simulink model "MMC_Rectifier_NLM_2018"  (R2023b)
settings: Solver=ode23t  StartTime=0.0  StopTime=3  RelTol=1e-3
libraries: spsIGBTDiodeLib x216, spsSeriesRLCBranchLib x117, spsVoltageMeasurementLib x110, spsCurrentMeasurementLib x7, slpidlib x6, spsThreePhaseVIMeasurementLib x2, spsGroundLib x1, spsPower3phInstantaneousLib x1, spsThreePhaseProgrammableVoltageSourceLib x1, spsThreePhaseSeriesRLCBranchLib x1, spspowerguiLib x1
(part 3 of 5)

== system MMC_Rectifier_NLM_2018/MMC  Rectifier/MMC1/MMC7 ==
  PWM : Inport
  IGBT/Diode : spsIGBTDiodeLib/IGBT//Diode  Ron=1e-3  Rs=1e5  Cs=inf  Measurements=off
  IGBT/Diode1 : spsIGBTDiodeLib/IGBT//Diode  Ron=1e-3  Rs=1e5  Cs=inf  Measurements=off
  Logical Operator : Logic  Inputs=1  AllPortsSameDT=off  OutDataTypeStr=boolean
  Logical Operator1 : Logic  Operator=NOT  Inputs=1  AllPortsSameDT=off  OutDataTypeStr=boolean
  Series RLC Branch : spsSeriesRLCBranchLib/Series RLC Branch  LConnTagsString=__new0  RConnTagsString=__new0  BranchType=C  Resistance=1  Inductance=1e-3  SetiL0=off  InitialCurrent=0  Capacitance=C0  Setx0=on  InitialVoltage=V0  Measurements=None
  Voltage Measurement : spsVoltageMeasurementLib/Voltage Measurement  PhasorSimulation=off  OutputType=Complex  PSBequivalent=0
  V+ : PMIOPort  Side=Left
  V- : PMIOPort  Port=2  Side=Left
  VC : Outport
  wires:
  Logical Operator1/1 -> IGBT/Diode1/1
  Voltage Measurement/1 -> VC/1
  Logical Operator/1 -> IGBT/Diode/1
  PWM/1 -> Logical Operator/1, Logical Operator1/1
  connections:
  Voltage Measurement/LConn1 -- Series RLC Branch/LConn1 -- IGBT/Diode/LConn1
  V+/RConn1 -- IGBT/Diode1/LConn1 -- IGBT/Diode/RConn1
  V-/RConn1 -- IGBT/Diode1/RConn1 -- Series RLC Branch/RConn1 -- Voltage Measurement/LConn2

== system MMC_Rectifier_NLM_2018/MMC  Rectifier/MMC1/MMC8 ==
  PWM : Inport
  IGBT/Diode : spsIGBTDiodeLib/IGBT//Diode  Ron=1e-3  Rs=1e5  Cs=inf  Measurements=off
  IGBT/Diode1 : spsIGBTDiodeLib/IGBT//Diode  Ron=1e-3  Rs=1e5  Cs=inf  Measurements=off
  Logical Operator : Logic  Inputs=1  AllPortsSameDT=off  OutDataTypeStr=boolean
  Logical Operator1 : Logic  Operator=NOT  Inputs=1  AllPortsSameDT=off  OutDataTypeStr=boolean
  Series RLC Branch : spsSeriesRLCBranchLib/Series RLC Branch  LConnTagsString=__new0  RConnTagsString=__new0  BranchType=C  Resistance=1  Inductance=1e-3  SetiL0=off  InitialCurrent=0  Capacitance=C0  Setx0=on  InitialVoltage=V0  Measurements=None
  Voltage Measurement : spsVoltageMeasurementLib/Voltage Measurement  PhasorSimulation=off  OutputType=Complex  PSBequivalent=0
  V+ : PMIOPort  Side=Left
  V- : PMIOPort  Port=2  Side=Left
  VC : Outport
  wires:
  Logical Operator1/1 -> IGBT/Diode1/1
  Voltage Measurement/1 -> VC/1
  Logical Operator/1 -> IGBT/Diode/1
  PWM/1 -> Logical Operator/1, Logical Operator1/1
  connections:
  Voltage Measurement/LConn1 -- Series RLC Branch/LConn1 -- IGBT/Diode/LConn1
  V+/RConn1 -- IGBT/Diode1/LConn1 -- IGBT/Diode/RConn1
  V-/RConn1 -- IGBT/Diode1/RConn1 -- Series RLC Branch/RConn1 -- Voltage Measurement/LConn2

== system MMC_Rectifier_NLM_2018/MMC  Rectifier/MMC1/MMC9 ==
  PWM : Inport
  IGBT/Diode : spsIGBTDiodeLib/IGBT//Diode  Ron=1e-3  Rs=1e5  Cs=inf  Measurements=off
  IGBT/Diode1 : spsIGBTDiodeLib/IGBT//Diode  Ron=1e-3  Rs=1e5  Cs=inf  Measurements=off
  Logical Operator : Logic  Inputs=1  AllPortsSameDT=off  OutDataTypeStr=boolean
  Logical Operator1 : Logic  Operator=NOT  Inputs=1  AllPortsSameDT=off  OutDataTypeStr=boolean
  Series RLC Branch : spsSeriesRLCBranchLib/Series RLC Branch  LConnTagsString=__new0  RConnTagsString=__new0  BranchType=C  Resistance=1  Inductance=1e-3  SetiL0=off  InitialCurrent=0  Capacitance=C0  Setx0=on  InitialVoltage=V0  Measurements=None
  Voltage Measurement : spsVoltageMeasurementLib/Voltage Measurement  PhasorSimulation=off  OutputType=Complex  PSBequivalent=0
  V+ : PMIOPort  Side=Left
  V- : PMIOPort  Port=2  Side=Left
  VC : Outport
  wires:
  PWM/1 -> Logical Operator1/1, Logical Operator/1
  Logical Operator/1 -> IGBT/Diode/1
  Voltage Measurement/1 -> VC/1
  Logical Operator1/1 -> IGBT/Diode1/1
  connections:
  Voltage Measurement/LConn2 -- Series RLC Branch/RConn1 -- IGBT/Diode1/RConn1 -- V-/RConn1
  IGBT/Diode/RConn1 -- IGBT/Diode1/LConn1 -- V+/RConn1
  IGBT/Diode/LConn1 -- Series RLC Branch/LConn1 -- Voltage Measurement/LConn1

== system MMC_Rectifier_NLM_2018/MMC  Rectifier/MMC2/MMC ==
  PWM : Inport
  IGBT/Diode : spsIGBTDiodeLib/IGBT//Diode  Ron=1e-3  Rs=1e5  Cs=inf  Measurements=off
  IGBT/Diode1 : spsIGBTDiodeLib/IGBT//Diode  Ron=1e-3  Rs=1e5  Cs=inf  Measurements=off
  Logical Operator : Logic  Inputs=1  AllPortsSameDT=off  OutDataTypeStr=boolean
  Logical Operator1 : Logic  Operator=NOT  Inputs=1  AllPortsSameDT=off  OutDataTypeStr=boolean
  Series RLC Branch : spsSeriesRLCBranchLib/Series RLC Branch  LConnTagsString=__new0  RConnTagsString=__new0  BranchType=C  Resistance=1  Inductance=1e-3  SetiL0=off  InitialCurrent=0  Capacitance=C0  Setx0=on  InitialVoltage=V0  Measurements=None
  Voltage Measurement : spsVoltageMeasurementLib/Voltage Measurement  PhasorSimulation=off  OutputType=Complex  PSBequivalent=0
  V+ : PMIOPort  Side=Left
  V- : PMIOPort  Port=2  Side=Left
  VC : Outport
  wires:
  PWM/1 -> Logical Operator1/1, Logical Operator/1
  Logical Operator/1 -> IGBT/Diode/1
  Voltage Measurement/1 -> VC/1
  Logical Operator1/1 -> IGBT/Diode1/1
  connections:
  Series RLC Branch/RConn1 -- Voltage Measurement/LConn2 -- V-/RConn1 -- IGBT/Diode1/RConn1
  IGBT/Diode1/LConn1 -- V+/RConn1 -- IGBT/Diode/RConn1
  Series RLC Branch/LConn1 -- Voltage Measurement/LConn1 -- IGBT/Diode/LConn1

== system MMC_Rectifier_NLM_2018/MMC  Rectifier/MMC2/MMC1 ==
  PWM : Inport
  IGBT/Diode : spsIGBTDiodeLib/IGBT//Diode  Ron=1e-3  Rs=1e5  Cs=inf  Measurements=off
  IGBT/Diode1 : spsIGBTDiodeLib/IGBT//Diode  Ron=1e-3  Rs=1e5  Cs=inf  Measurements=off
  Logical Operator : Logic  Inputs=1  AllPortsSameDT=off  OutDataTypeStr=boolean
  Logical Operator1 : Logic  Operator=NOT  Inputs=1  AllPortsSameDT=off  OutDataTypeStr=boolean
  Series RLC Branch : spsSeriesRLCBranchLib/Series RLC Branch  LConnTagsString=__new0  RConnTagsString=__new0  BranchType=C  Resistance=1  Inductance=1e-3  SetiL0=off  InitialCurrent=0  Capacitance=C0  Setx0=on  InitialVoltage=V0  Measurements=None
  Voltage Measurement : spsVoltageMeasurementLib/Voltage Measurement  PhasorSimulation=off  OutputType=Complex  PSBequivalent=0
  V+ : PMIOPort  Side=Left
  V- : PMIOPort  Port=2  Side=Left
  VC : Outport
  wires:
  Logical Operator1/1 -> IGBT/Diode1/1
  Voltage Measurement/1 -> VC/1
  Logical Operator/1 -> IGBT/Diode/1
  PWM/1 -> Logical Operator/1, Logical Operator1/1
  connections:
  Voltage Measurement/LConn1 -- Series RLC Branch/LConn1 -- IGBT/Diode/LConn1
  V+/RConn1 -- IGBT/Diode1/LConn1 -- IGBT/Diode/RConn1
  V-/RConn1 -- IGBT/Diode1/RConn1 -- Series RLC Branch/RConn1 -- Voltage Measurement/LConn2

== system MMC_Rectifier_NLM_2018/MMC  Rectifier/MMC2/MMC10 ==
  PWM : Inport
  IGBT/Diode : spsIGBTDiodeLib/IGBT//Diode  Ron=1e-3  Rs=1e5  Cs=inf  Measurements=off
  IGBT/Diode1 : spsIGBTDiodeLib/IGBT//Diode  Ron=1e-3  Rs=1e5  Cs=inf  Measurements=off
  Logical Operator : Logic  Inputs=1  AllPortsSameDT=off  OutDataTypeStr=boolean
  Logical Operator1 : Logic  Operator=NOT  Inputs=1  AllPortsSameDT=off  OutDataTypeStr=boolean
  Series RLC Branch : spsSeriesRLCBranchLib/Series RLC Branch  LConnTagsString=__new0  RConnTagsString=__new0  BranchType=C  Resistance=1  Inductance=1e-3  SetiL0=off  InitialCurrent=0  Capacitance=C0  Setx0=on  InitialVoltage=V0  Measurements=None
  Voltage Measurement : spsVoltageMeasurementLib/Voltage Measurement  PhasorSimulation=off  OutputType=Complex  PSBequivalent=0
  V+ : PMIOPort  Side=Left
  V- : PMIOPort  Port=2  Side=Left
  VC : Outport
  wires:
  Logical Operator1/1 -> IGBT/Diode1/1
  Voltage Measurement/1 -> VC/1
  Logical Operator/1 -> IGBT/Diode/1
  PWM/1 -> Logical Operator/1, Logical Operator1/1
  connections:
  Voltage Measurement/LConn1 -- Series RLC Branch/LConn1 -- IGBT/Diode/LConn1
  V+/RConn1 -- IGBT/Diode1/LConn1 -- IGBT/Diode/RConn1
  V-/RConn1 -- IGBT/Diode1/RConn1 -- Series RLC Branch/RConn1 -- Voltage Measurement/LConn2

== system MMC_Rectifier_NLM_2018/MMC  Rectifier/MMC2/MMC11 ==
  PWM : Inport
  IGBT/Diode : spsIGBTDiodeLib/IGBT//Diode  Ron=1e-3  Rs=1e5  Cs=inf  Measurements=off
  IGBT/Diode1 : spsIGBTDiodeLib/IGBT//Diode  Ron=1e-3  Rs=1e5  Cs=inf  Measurements=off
  Logical Operator : Logic  Inputs=1  AllPortsSameDT=off  OutDataTypeStr=boolean
  Logical Operator1 : Logic  Operator=NOT  Inputs=1  AllPortsSameDT=off  OutDataTypeStr=boolean
  Series RLC Branch : spsSeriesRLCBranchLib/Series RLC Branch  LConnTagsString=__new0  RConnTagsString=__new0  BranchType=C  Resistance=1  Inductance=1e-3  SetiL0=off  InitialCurrent=0  Capacitance=C0  Setx0=on  InitialVoltage=V0  Measurements=None
  Voltage Measurement : spsVoltageMeasurementLib/Voltage Measurement  PhasorSimulation=off  OutputType=Complex  PSBequivalent=0
  V+ : PMIOPort  Side=Left
  V- : PMIOPort  Port=2  Side=Left
  VC : Outport
  wires:
  PWM/1 -> Logical Operator1/1, Logical Operator/1
  Logical Operator/1 -> IGBT/Diode/1
  Voltage Measurement/1 -> VC/1
  Logical Operator1/1 -> IGBT/Diode1/1
  connections:
  Voltage Measurement/LConn2 -- Series RLC Branch/RConn1 -- IGBT/Diode1/RConn1 -- V-/RConn1
  IGBT/Diode/RConn1 -- IGBT/Diode1/LConn1 -- V+/RConn1
  IGBT/Diode/LConn1 -- Series RLC Branch/LConn1 -- Voltage Measurement/LConn1

== system MMC_Rectifier_NLM_2018/MMC  Rectifier/MMC2/MMC12 ==
  PWM : Inport
  IGBT/Diode : spsIGBTDiodeLib/IGBT//Diode  Ron=1e-3  Rs=1e5  Cs=inf  Measurements=off
  IGBT/Diode1 : spsIGBTDiodeLib/IGBT//Diode  Ron=1e-3  Rs=1e5  Cs=inf  Measurements=off
  Logical Operator : Logic  Inputs=1  AllPortsSameDT=off  OutDataTypeStr=boolean
  Logical Operator1 : Logic  Operator=NOT  Inputs=1  AllPortsSameDT=off  OutDataTypeStr=boolean
  Series RLC Branch : spsSeriesRLCBranchLib/Series RLC Branch  LConnTagsString=__new0  RConnTagsString=__new0  BranchType=C  Resistance=1  Inductance=1e-3  SetiL0=off  InitialCurrent=0  Capacitance=C0  Setx0=on  InitialVoltage=V0  Measurements=None
  Voltage Measurement : spsVoltageMeasurementLib/Voltage Measurement  PhasorSimulation=off  OutputType=Complex  PSBequivalent=0
  V+ : PMIOPort  Side=Left
  V- : PMIOPort  Port=2  Side=Left
  VC : Outport
  wires:
  PWM/1 -> Logical Operator1/1, Logical Operator/1
  Logical Operator/1 -> IGBT/Diode/1
  Voltage Measurement/1 -> VC/1
  Logical Operator1/1 -> IGBT/Diode1/1
  connections:
  Voltage Measurement/LConn2 -- Series RLC Branch/RConn1 -- IGBT/Diode1/RConn1 -- V-/RConn1
  IGBT/Diode/RConn1 -- IGBT/Diode1/LConn1 -- V+/RConn1
  IGBT/Diode/LConn1 -- Series RLC Branch/LConn1 -- Voltage Measurement/LConn1

== system MMC_Rectifier_NLM_2018/MMC  Rectifier/MMC2/MMC13 ==
  PWM : Inport
  IGBT/Diode : spsIGBTDiodeLib/IGBT//Diode  Ron=1e-3  Rs=1e5  Cs=inf  Measurements=off
  IGBT/Diode1 : spsIGBTDiodeLib/IGBT//Diode  Ron=1e-3  Rs=1e5  Cs=inf  Measurements=off
  Logical Operator : Logic  Inputs=1  AllPortsSameDT=off  OutDataTypeStr=boolean
  Logical Operator1 : Logic  Operator=NOT  Inputs=1  AllPortsSameDT=off  OutDataTypeStr=boolean
  Series RLC Branch : spsSeriesRLCBranchLib/Series RLC Branch  LConnTagsString=__new0  RConnTagsString=__new0  BranchType=C  Resistance=1  Inductance=1e-3  SetiL0=off  InitialCurrent=0  Capacitance=C0  Setx0=on  InitialVoltage=V0  Measurements=None
  Voltage Measurement : spsVoltageMeasurementLib/Voltage Measurement  PhasorSimulation=off  OutputType=Complex  PSBequivalent=0
  V+ : PMIOPort  Side=Left
  V- : PMIOPort  Port=2  Side=Left
  VC : Outport
  wires:
  Logical Operator1/1 -> IGBT/Diode1/1
  Voltage Measurement/1 -> VC/1
  Logical Operator/1 -> IGBT/Diode/1
  PWM/1 -> Logical Operator/1, Logical Operator1/1
  connections:
  Voltage Measurement/LConn1 -- Series RLC Branch/LConn1 -- IGBT/Diode/LConn1
  V+/RConn1 -- IGBT/Diode1/LConn1 -- IGBT/Diode/RConn1
  V-/RConn1 -- IGBT/Diode1/RConn1 -- Series RLC Branch/RConn1 -- Voltage Measurement/LConn2

== system MMC_Rectifier_NLM_2018/MMC  Rectifier/MMC2/MMC14 ==
  PWM : Inport
  IGBT/Diode : spsIGBTDiodeLib/IGBT//Diode  Ron=1e-3  Rs=1e5  Cs=inf  Measurements=off
  IGBT/Diode1 : spsIGBTDiodeLib/IGBT//Diode  Ron=1e-3  Rs=1e5  Cs=inf  Measurements=off
  Logical Operator : Logic  Inputs=1  AllPortsSameDT=off  OutDataTypeStr=boolean
  Logical Operator1 : Logic  Operator=NOT  Inputs=1  AllPortsSameDT=off  OutDataTypeStr=boolean
  Series RLC Branch : spsSeriesRLCBranchLib/Series RLC Branch  LConnTagsString=__new0  RConnTagsString=__new0  BranchType=C  Resistance=1  Inductance=1e-3  SetiL0=off  InitialCurrent=0  Capacitance=C0  Setx0=on  InitialVoltage=V0  Measurements=None
  Voltage Measurement : spsVoltageMeasurementLib/Voltage Measurement  PhasorSimulation=off  OutputType=Complex  PSBequivalent=0
  V+ : PMIOPort  Side=Left
  V- : PMIOPort  Port=2  Side=Left
  VC : Outport
  wires:
  PWM/1 -> Logical Operator1/1, Logical Operator/1
  Logical Operator/1 -> IGBT/Diode/1
  Voltage Measurement/1 -> VC/1
  Logical Operator1/1 -> IGBT/Diode1/1
  connections:
  Series RLC Branch/RConn1 -- Voltage Measurement/LConn2 -- V-/RConn1 -- IGBT/Diode1/RConn1
  IGBT/Diode1/LConn1 -- V+/RConn1 -- IGBT/Diode/RConn1
  Series RLC Branch/LConn1 -- Voltage Measurement/LConn1 -- IGBT/Diode/LConn1

== system MMC_Rectifier_NLM_2018/MMC  Rectifier/MMC2/MMC15 ==
  PWM : Inport
  IGBT/Diode : spsIGBTDiodeLib/IGBT//Diode  Ron=1e-3  Rs=1e5  Cs=inf  Measurements=off
  IGBT/Diode1 : spsIGBTDiodeLib/IGBT//Diode  Ron=1e-3  Rs=1e5  Cs=inf  Measurements=off
  Logical Operator : Logic  Inputs=1  AllPortsSameDT=off  OutDataTypeStr=boolean
  Logical Operator1 : Logic  Operator=NOT  Inputs=1  AllPortsSameDT=off  OutDataTypeStr=boolean
  Series RLC Branch : spsSeriesRLCBranchLib/Series RLC Branch  LConnTagsString=__new0  RConnTagsString=__new0  BranchType=C  Resistance=1  Inductance=1e-3  SetiL0=off  InitialCurrent=0  Capacitance=C0  Setx0=on  InitialVoltage=V0  Measurements=None
  Voltage Measurement : spsVoltageMeasurementLib/Voltage Measurement  PhasorSimulation=off  OutputType=Complex  PSBequivalent=0
  V+ : PMIOPort  Side=Left
  V- : PMIOPort  Port=2  Side=Left
  VC : Outport
  wires:
  Logical Operator1/1 -> IGBT/Diode1/1
  Voltage Measurement/1 -> VC/1
  Logical Operator/1 -> IGBT/Diode/1
  PWM/1 -> Logical Operator/1, Logical Operator1/1
  connections:
  Voltage Measurement/LConn1 -- Series RLC Branch/LConn1 -- IGBT/Diode/LConn1
  V+/RConn1 -- IGBT/Diode1/LConn1 -- IGBT/Diode/RConn1
  V-/RConn1 -- IGBT/Diode1/RConn1 -- Series RLC Branch/RConn1 -- Voltage Measurement/LConn2

== system MMC_Rectifier_NLM_2018/MMC  Rectifier/MMC2/MMC16 ==
  PWM : Inport
  IGBT/Diode : spsIGBTDiodeLib/IGBT//Diode  Ron=1e-3  Rs=1e5  Cs=inf  Measurements=off
  IGBT/Diode1 : spsIGBTDiodeLib/IGBT//Diode  Ron=1e-3  Rs=1e5  Cs=inf  Measurements=off
  Logical Operator : Logic  Inputs=1  AllPortsSameDT=off  OutDataTypeStr=boolean
  Logical Operator1 : Logic  Operator=NOT  Inputs=1  AllPortsSameDT=off  OutDataTypeStr=boolean
  Series RLC Branch : spsSeriesRLCBranchLib/Series RLC Branch  LConnTagsString=__new0  RConnTagsString=__new0  BranchType=C  Resistance=1  Inductance=1e-3  SetiL0=off  InitialCurrent=0  Capacitance=C0  Setx0=on  InitialVoltage=V0  Measurements=None
  Voltage Measurement : spsVoltageMeasurementLib/Voltage Measurement  PhasorSimulation=off  OutputType=Complex  PSBequivalent=0
  V+ : PMIOPort  Side=Left
  V- : PMIOPort  Port=2  Side=Left
  VC : Outport
  wires:
  Logical Operator1/1 -> IGBT/Diode1/1
  Voltage Measurement/1 -> VC/1
  Logical Operator/1 -> IGBT/Diode/1
  PWM/1 -> Logical Operator/1, Logical Operator1/1
  connections:
  Voltage Measurement/LConn1 -- Series RLC Branch/LConn1 -- IGBT/Diode/LConn1
  V+/RConn1 -- IGBT/Diode1/LConn1 -- IGBT/Diode/RConn1
  V-/RConn1 -- IGBT/Diode1/RConn1 -- Series RLC Branch/RConn1 -- Voltage Measurement/LConn2

== system MMC_Rectifier_NLM_2018/MMC  Rectifier/MMC2/MMC17 ==
  PWM : Inport
  IGBT/Diode : spsIGBTDiodeLib/IGBT//Diode  Ron=1e-3  Rs=1e5  Cs=inf  Measurements=off
  IGBT/Diode1 : spsIGBTDiodeLib/IGBT//Diode  Ron=1e-3  Rs=1e5  Cs=inf  Measurements=off
  Logical Operator : Logic  Inputs=1  AllPortsSameDT=off  OutDataTypeStr=boolean
  Logical Operator1 : Logic  Operator=NOT  Inputs=1  AllPortsSameDT=off  OutDataTypeStr=boolean
  Series RLC Branch : spsSeriesRLCBranchLib/Series RLC Branch  LConnTagsString=__new0  RConnTagsString=__new0  BranchType=C  Resistance=1  Inductance=1e-3  SetiL0=off  InitialCurrent=0  Capacitance=C0  Setx0=on  InitialVoltage=V0  Measurements=None
  Voltage Measurement : spsVoltageMeasurementLib/Voltage Measurement  PhasorSimulation=off  OutputType=Complex  PSBequivalent=0
  V+ : PMIOPort  Side=Left
  V- : PMIOPort  Port=2  Side=Left
  VC : Outport
  wires:
  PWM/1 -> Logical Operator1/1, Logical Operator/1
  Logical Operator/1 -> IGBT/Diode/1
  Voltage Measurement/1 -> VC/1
  Logical Operator1/1 -> IGBT/Diode1/1
  connections:
  Voltage Measurement/LConn2 -- Series RLC Branch/RConn1 -- IGBT/Diode1/RConn1 -- V-/RConn1
  IGBT/Diode/RConn1 -- IGBT/Diode1/LConn1 -- V+/RConn1
  IGBT/Diode/LConn1 -- Series RLC Branch/LConn1 -- Voltage Measurement/LConn1

== system MMC_Rectifier_NLM_2018/MMC  Rectifier/MMC2/MMC2 ==
  PWM : Inport
  IGBT/Diode : spsIGBTDiodeLib/IGBT//Diode  Ron=1e-3  Rs=1e5  Cs=inf  Measurements=off
  IGBT/Diode1 : spsIGBTDiodeLib/IGBT//Diode  Ron=1e-3  Rs=1e5  Cs=inf  Measurements=off
  Logical Operator : Logic  Inputs=1  AllPortsSameDT=off  OutDataTypeStr=boolean
  Logical Operator1 : Logic  Operator=NOT  Inputs=1  AllPortsSameDT=off  OutDataTypeStr=boolean
  Series RLC Branch : spsSeriesRLCBranchLib/Series RLC Branch  LConnTagsString=__new0  RConnTagsString=__new0  BranchType=C  Resistance=1  Inductance=1e-3  SetiL0=off  InitialCurrent=0  Capacitance=C0  Setx0=on  InitialVoltage=V0  Measurements=None
  Voltage Measurement : spsVoltageMeasurementLib/Voltage Measurement  PhasorSimulation=off  OutputType=Complex  PSBequivalent=0
  V+ : PMIOPort  Side=Left
  V- : PMIOPort  Port=2  Side=Left
  VC : Outport
  wires:
  Logical Operator1/1 -> IGBT/Diode1/1
  Voltage Measurement/1 -> VC/1
  Logical Operator/1 -> IGBT/Diode/1
  PWM/1 -> Logical Operator/1, Logical Operator1/1
  connections:
  Voltage Measurement/LConn1 -- Series RLC Branch/LConn1 -- IGBT/Diode/LConn1
  V+/RConn1 -- IGBT/Diode1/LConn1 -- IGBT/Diode/RConn1
  V-/RConn1 -- IGBT/Diode1/RConn1 -- Series RLC Branch/RConn1 -- Voltage Measurement/LConn2

== system MMC_Rectifier_NLM_2018/MMC  Rectifier/MMC2/MMC3 ==
  PWM : Inport
  IGBT/Diode : spsIGBTDiodeLib/IGBT//Diode  Ron=1e-3  Rs=1e5  Cs=inf  Measurements=off
  IGBT/Diode1 : spsIGBTDiodeLib/IGBT//Diode  Ron=1e-3  Rs=1e5  Cs=inf  Measurements=off
  Logical Operator : Logic  Inputs=1  AllPortsSameDT=off  OutDataTypeStr=boolean
  Logical Operator1 : Logic  Operator=NOT  Inputs=1  AllPortsSameDT=off  OutDataTypeStr=boolean
  Series RLC Branch : spsSeriesRLCBranchLib/Series RLC Branch  LConnTagsString=__new0  RConnTagsString=__new0  BranchType=C  Resistance=1  Inductance=1e-3  SetiL0=off  InitialCurrent=0  Capacitance=C0  Setx0=on  InitialVoltage=V0  Measurements=None
  Voltage Measurement : spsVoltageMeasurementLib/Voltage Measurement  PhasorSimulation=off  OutputType=Complex  PSBequivalent=0
  V+ : PMIOPort  Side=Left
  V- : PMIOPort  Port=2  Side=Left
  VC : Outport
  wires:
  PWM/1 -> Logical Operator1/1, Logical Operator/1
  Logical Operator/1 -> IGBT/Diode/1
  Voltage Measurement/1 -> VC/1
  Logical Operator1/1 -> IGBT/Diode1/1
  connections:
  Voltage Measurement/LConn2 -- Series RLC Branch/RConn1 -- IGBT/Diode1/RConn1 -- V-/RConn1
  IGBT/Diode/RConn1 -- IGBT/Diode1/LConn1 -- V+/RConn1
  IGBT/Diode/LConn1 -- Series RLC Branch/LConn1 -- Voltage Measurement/LConn1

== system MMC_Rectifier_NLM_2018/MMC  Rectifier/MMC2/MMC4 ==
  PWM : Inport
  IGBT/Diode : spsIGBTDiodeLib/IGBT//Diode  Ron=1e-3  Rs=1e5  Cs=inf  Measurements=off
  IGBT/Diode1 : spsIGBTDiodeLib/IGBT//Diode  Ron=1e-3  Rs=1e5  Cs=inf  Measurements=off
  Logical Operator : Logic  Inputs=1  AllPortsSameDT=off  OutDataTypeStr=boolean
  Logical Operator1 : Logic  Operator=NOT  Inputs=1  AllPortsSameDT=off  OutDataTypeStr=boolean
  Series RLC Branch : spsSeriesRLCBranchLib/Series RLC Branch  LConnTagsString=__new0  RConnTagsString=__new0  BranchType=C  Resistance=1  Inductance=1e-3  SetiL0=off  InitialCurrent=0  Capacitance=C0  Setx0=on  InitialVoltage=V0  Measurements=None
  Voltage Measurement : spsVoltageMeasurementLib/Voltage Measurement  PhasorSimulation=off  OutputType=Complex  PSBequivalent=0
  V+ : PMIOPort  Side=Left
  V- : PMIOPort  Port=2  Side=Left
  VC : Outport
  wires:
  PWM/1 -> Logical Operator1/1, Logical Operator/1
  Logical Operator/1 -> IGBT/Diode/1
  Voltage Measurement/1 -> VC/1
  Logical Operator1/1 -> IGBT/Diode1/1
  connections:
  Voltage Measurement/LConn2 -- Series RLC Branch/RConn1 -- IGBT/Diode1/RConn1 -- V-/RConn1
  IGBT/Diode/RConn1 -- IGBT/Diode1/LConn1 -- V+/RConn1
  IGBT/Diode/LConn1 -- Series RLC Branch/LConn1 -- Voltage Measurement/LConn1

== system MMC_Rectifier_NLM_2018/MMC  Rectifier/MMC2/MMC5 ==
  PWM : Inport
  IGBT/Diode : spsIGBTDiodeLib/IGBT//Diode  Ron=1e-3  Rs=1e5  Cs=inf  Measurements=off
  IGBT/Diode1 : spsIGBTDiodeLib/IGBT//Diode  Ron=1e-3  Rs=1e5  Cs=inf  Measurements=off
  Logical Operator : Logic  Inputs=1  AllPortsSameDT=off  OutDataTypeStr=boolean
  Logical Operator1 : Logic  Operator=NOT  Inputs=1  AllPortsSameDT=off  OutDataTypeStr=boolean
  Series RLC Branch : spsSeriesRLCBranchLib/Series RLC Branch  LConnTagsString=__new0  RConnTagsString=__new0  BranchType=C  Resistance=1  Inductance=1e-3  SetiL0=off  InitialCurrent=0  Capacitance=C0  Setx0=on  InitialVoltage=V0  Measurements=None
  Voltage Measurement : spsVoltageMeasurementLib/Voltage Measurement  PhasorSimulation=off  OutputType=Complex  PSBequivalent=0
  V+ : PMIOPort  Side=Left
  V- : PMIOPort  Port=2  Side=Left
  VC : Outport
  wires:
  Logical Operator1/1 -> IGBT/Diode1/1
  Voltage Measurement/1 -> VC/1
  Logical Operator/1 -> IGBT/Diode/1
  PWM/1 -> Logical Operator/1, Logical Operator1/1
  connections:
  Voltage Measurement/LConn1 -- Series RLC Branch/LConn1 -- IGBT/Diode/LConn1
  V+/RConn1 -- IGBT/Diode1/LConn1 -- IGBT/Diode/RConn1
  V-/RConn1 -- IGBT/Diode1/RConn1 -- Series RLC Branch/RConn1 -- Voltage Measurement/LConn2

== system MMC_Rectifier_NLM_2018/MMC  Rectifier/MMC2/MMC6 ==
  PWM : Inport
  IGBT/Diode : spsIGBTDiodeLib/IGBT//Diode  Ron=1e-3  Rs=1e5  Cs=inf  Measurements=off
  IGBT/Diode1 : spsIGBTDiodeLib/IGBT//Diode  Ron=1e-3  Rs=1e5  Cs=inf  Measurements=off
  Logical Operator : Logic  Inputs=1  AllPortsSameDT=off  OutDataTypeStr=boolean
  Logical Operator1 : Logic  Operator=NOT  Inputs=1  AllPortsSameDT=off  OutDataTypeStr=boolean
  Series RLC Branch : spsSeriesRLCBranchLib/Series RLC Branch  LConnTagsString=__new0  RConnTagsString=__new0  BranchType=C  Resistance=1  Inductance=1e-3  SetiL0=off  InitialCurrent=0  Capacitance=C0  Setx0=on  InitialVoltage=V0  Measurements=None
  Voltage Measurement : spsVoltageMeasurementLib/Voltage Measurement  PhasorSimulation=off  OutputType=Complex  PSBequivalent=0
  V+ : PMIOPort  Side=Left
  V- : PMIOPort  Port=2  Side=Left
  VC : Outport
  wires:
  Logical Operator1/1 -> IGBT/Diode1/1
  Voltage Measurement/1 -> VC/1
  Logical Operator/1 -> IGBT/Diode/1
  PWM/1 -> Logical Operator/1, Logical Operator1/1
  connections:
  IGBT/Diode/LConn1 -- Voltage Measurement/LConn1 -- Series RLC Branch/LConn1
  IGBT/Diode/RConn1 -- V+/RConn1 -- IGBT/Diode1/LConn1
  IGBT/Diode1/RConn1 -- V-/RConn1 -- Voltage Measurement/LConn2 -- Series RLC Branch/RConn1

== system MMC_Rectifier_NLM_2018/MMC  Rectifier/MMC2/MMC7 ==
  PWM : Inport
  IGBT/Diode : spsIGBTDiodeLib/IGBT//Diode  Ron=1e-3  Rs=1e5  Cs=inf  Measurements=off
  IGBT/Diode1 : spsIGBTDiodeLib/IGBT//Diode  Ron=1e-3  Rs=1e5  Cs=inf  Measurements=off
  Logical Operator : Logic  Inputs=1  AllPortsSameDT=off  OutDataTypeStr=boolean
  Logical Operator1 : Logic  Operator=NOT  Inputs=1  AllPortsSameDT=off  OutDataTypeStr=boolean
  Series RLC Branch : spsSeriesRLCBranchLib/Series RLC Branch  LConnTagsString=__new0  RConnTagsString=__new0  BranchType=C  Resistance=1  Inductance=1e-3  SetiL0=off  InitialCurrent=0  Capacitance=C0  Setx0=on  InitialVoltage=V0  Measurements=None
  Voltage Measurement : spsVoltageMeasurementLib/Voltage Measurement  PhasorSimulation=off  OutputType=Complex  PSBequivalent=0
  V+ : PMIOPort  Side=Left
  V- : PMIOPort  Port=2  Side=Left
  VC : Outport
  wires:
  PWM/1 -> Logical Operator1/1, Logical Operator/1
  Logical Operator/1 -> IGBT/Diode/1
  Voltage Measurement/1 -> VC/1
  Logical Operator1/1 -> IGBT/Diode1/1
  connections:
  Voltage Measurement/LConn2 -- Series RLC Branch/RConn1 -- IGBT/Diode1/RConn1 -- V-/RConn1
  IGBT/Diode/RConn1 -- IGBT/Diode1/LConn1 -- V+/RConn1
  IGBT/Diode/LConn1 -- Series RLC Branch/LConn1 -- Voltage Measurement/LConn1

== system MMC_Rectifier_NLM_2018/MMC  Rectifier/MMC2/MMC8 ==
  PWM : Inport
  IGBT/Diode : spsIGBTDiodeLib/IGBT//Diode  Ron=1e-3  Rs=1e5  Cs=inf  Measurements=off
  IGBT/Diode1 : spsIGBTDiodeLib/IGBT//Diode  Ron=1e-3  Rs=1e5  Cs=inf  Measurements=off
  Logical Operator : Logic  Inputs=1  AllPortsSameDT=off  OutDataTypeStr=boolean
  Logical Operator1 : Logic  Operator=NOT  Inputs=1  AllPortsSameDT=off  OutDataTypeStr=boolean
  Series RLC Branch : spsSeriesRLCBranchLib/Series RLC Branch  LConnTagsString=__new0  RConnTagsString=__new0  BranchType=C  Resistance=1  Inductance=1e-3  SetiL0=off  InitialCurrent=0  Capacitance=C0  Setx0=on  InitialVoltage=V0  Measurements=None
  Voltage Measurement : spsVoltageMeasurementLib/Voltage Measurement  PhasorSimulation=off  OutputType=Complex  PSBequivalent=0
  V+ : PMIOPort  Side=Left
  V- : PMIOPort  Port=2  Side=Left
  VC : Outport
  wires:
  PWM/1 -> Logical Operator1/1, Logical Operator/1
  Logical Operator/1 -> IGBT/Diode/1
  Voltage Measurement/1 -> VC/1
  Logical Operator1/1 -> IGBT/Diode1/1
  connections:
  Voltage Measurement/LConn2 -- Series RLC Branch/RConn1 -- IGBT/Diode1/RConn1 -- V-/RConn1
  IGBT/Diode/RConn1 -- IGBT/Diode1/LConn1 -- V+/RConn1
  IGBT/Diode/LConn1 -- Series RLC Branch/LConn1 -- Voltage Measurement/LConn1

== system MMC_Rectifier_NLM_2018/MMC  Rectifier/MMC2/MMC9 ==
  PWM : Inport
  IGBT/Diode : spsIGBTDiodeLib/IGBT//Diode  Ron=1e-3  Rs=1e5  Cs=inf  Measurements=off
  IGBT/Diode1 : spsIGBTDiodeLib/IGBT//Diode  Ron=1e-3  Rs=1e5  Cs=inf  Measurements=off
  Logical Operator : Logic  Inputs=1  AllPortsSameDT=off  OutDataTypeStr=boolean
  Logical Operator1 : Logic  Operator=NOT  Inputs=1  AllPortsSameDT=off  OutDataTypeStr=boolean
  Series RLC Branch : spsSeriesRLCBranchLib/Series RLC Branch  LConnTagsString=__new0  RConnTagsString=__new0  BranchType=C  Resistance=1  Inductance=1e-3  SetiL0=off  InitialCurrent=0  Capacitance=C0  Setx0=on  InitialVoltage=V0  Measurements=None
  Voltage Measurement : spsVoltageMeasurementLib/Voltage Measurement  PhasorSimulation=off  OutputType=Complex  PSBequivalent=0
  V+ : PMIOPort  Side=Left
  V- : PMIOPort  Port=2  Side=Left
  VC : Outport
  wires:
  Logical Operator1/1 -> IGBT/Diode1/1
  Voltage Measurement/1 -> VC/1
  Logical Operator/1 -> IGBT/Diode/1
  PWM/1 -> Logical Operator/1, Logical Operator1/1
  connections:
  Voltage Measurement/LConn1 -- Series RLC Branch/LConn1 -- IGBT/Diode/LConn1
  V+/RConn1 -- IGBT/Diode1/LConn1 -- IGBT/Diode/RConn1
  V-/RConn1 -- IGBT/Diode1/RConn1 -- Series RLC Branch/RConn1 -- Voltage Measurement/LConn2

== system MMC_Rectifier_NLM_2018/MMC  Rectifier/MMC3/MMC ==
  PWM : Inport
  IGBT/Diode : spsIGBTDiodeLib/IGBT//Diode  Ron=1e-3  Rs=1e5  Cs=inf  Measurements=off
  IGBT/Diode1 : spsIGBTDiodeLib/IGBT//Diode  Ron=1e-3  Rs=1e5  Cs=inf  Measurements=off
  Logical Operator : Logic  Inputs=1  AllPortsSameDT=off  OutDataTypeStr=boolean
  Logical Operator1 : Logic  Operator=NOT  Inputs=1  AllPortsSameDT=off  OutDataTypeStr=boolean
  Series RLC Branch : spsSeriesRLCBranchLib/Series RLC Branch  LConnTagsString=__new0  RConnTagsString=__new0  BranchType=C  Resistance=1  Inductance=1e-3  SetiL0=off  InitialCurrent=0  Capacitance=C0  Setx0=on  InitialVoltage=V0  Measurements=None
  Voltage Measurement : spsVoltageMeasurementLib/Voltage Measurement  PhasorSimulation=off  OutputType=Complex  PSBequivalent=0
  V+ : PMIOPort  Side=Left
  V- : PMIOPort  Port=2  Side=Left
  VC : Outport
  wires:
  Logical Operator1/1 -> IGBT/Diode1/1
  Voltage Measurement/1 -> VC/1
  Logical Operator/1 -> IGBT/Diode/1
  PWM/1 -> Logical Operator/1, Logical Operator1/1
  connections:
  IGBT/Diode/LConn1 -- Voltage Measurement/LConn1 -- Series RLC Branch/LConn1
  IGBT/Diode/RConn1 -- V+/RConn1 -- IGBT/Diode1/LConn1
  IGBT/Diode1/RConn1 -- V-/RConn1 -- Voltage Measurement/LConn2 -- Series RLC Branch/RConn1

== system MMC_Rectifier_NLM_2018/MMC  Rectifier/MMC3/MMC1 ==
  PWM : Inport
  IGBT/Diode : spsIGBTDiodeLib/IGBT//Diode  Ron=1e-3  Rs=1e5  Cs=inf  Measurements=off
  IGBT/Diode1 : spsIGBTDiodeLib/IGBT//Diode  Ron=1e-3  Rs=1e5  Cs=inf  Measurements=off
  Logical Operator : Logic  Inputs=1  AllPortsSameDT=off  OutDataTypeStr=boolean
  Logical Operator1 : Logic  Operator=NOT  Inputs=1  AllPortsSameDT=off  OutDataTypeStr=boolean
  Series RLC Branch : spsSeriesRLCBranchLib/Series RLC Branch  LConnTagsString=__new0  RConnTagsString=__new0  BranchType=C  Resistance=1  Inductance=1e-3  SetiL0=off  InitialCurrent=0  Capacitance=C0  Setx0=on  InitialVoltage=V0  Measurements=None
  Voltage Measurement : spsVoltageMeasurementLib/Voltage Measurement  PhasorSimulation=off  OutputType=Complex  PSBequivalent=0
  V+ : PMIOPort  Side=Left
  V- : PMIOPort  Port=2  Side=Left
  VC : Outport
  wires:
  PWM/1 -> Logical Operator1/1, Logical Operator/1
  Logical Operator/1 -> IGBT/Diode/1
  Voltage Measurement/1 -> VC/1
  Logical Operator1/1 -> IGBT/Diode1/1
  connections:
  Voltage Measurement/LConn2 -- Series RLC Branch/RConn1 -- IGBT/Diode1/RConn1 -- V-/RConn1
  IGBT/Diode/RConn1 -- IGBT/Diode1/LConn1 -- V+/RConn1
  IGBT/Diode/LConn1 -- Series RLC Branch/LConn1 -- Voltage Measurement/LConn1

== system MMC_Rectifier_NLM_2018/MMC  Rectifier/MMC3/MMC10 ==
  PWM : Inport
  IGBT/Diode : spsIGBTDiodeLib/IGBT//Diode  Ron=1e-3  Rs=1e5  Cs=inf  Measurements=off
  IGBT/Diode1 : spsIGBTDiodeLib/IGBT//Diode  Ron=1e-3  Rs=1e5  Cs=inf  Measurements=off
  Logical Operator : Logic  Inputs=1  AllPortsSameDT=off  OutDataTypeStr=boolean
  Logical Operator1 : Logic  Operator=NOT  Inputs=1  AllPortsSameDT=off  OutDataTypeStr=boolean
  Series RLC Branch : spsSeriesRLCBranchLib/Series RLC Branch  LConnTagsString=__new0  RConnTagsString=__new0  BranchType=C  Resistance=1  Inductance=1e-3  SetiL0=off  InitialCurrent=0  Capacitance=C0  Setx0=on  InitialVoltage=V0  Measurements=None
  Voltage Measurement : spsVoltageMeasurementLib/Voltage Measurement  PhasorSimulation=off  OutputType=Complex  PSBequivalent=0
  V+ : PMIOPort  Side=Left
  V- : PMIOPort  Port=2  Side=Left
  VC : Outport
  wires:
  PWM/1 -> Logical Operator1/1, Logical Operator/1
  Logical Operator/1 -> IGBT/Diode/1
  Voltage Measurement/1 -> VC/1
  Logical Operator1/1 -> IGBT/Diode1/1
  connections:
  Voltage Measurement/LConn2 -- Series RLC Branch/RConn1 -- IGBT/Diode1/RConn1 -- V-/RConn1
  IGBT/Diode/RConn1 -- IGBT/Diode1/LConn1 -- V+/RConn1
  IGBT/Diode/LConn1 -- Series RLC Branch/LConn1 -- Voltage Measurement/LConn1

== system MMC_Rectifier_NLM_2018/MMC  Rectifier/MMC3/MMC11 ==
  PWM : Inport
  IGBT/Diode : spsIGBTDiodeLib/IGBT//Diode  Ron=1e-3  Rs=1e5  Cs=inf  Measurements=off
  IGBT/Diode1 : spsIGBTDiodeLib/IGBT//Diode  Ron=1e-3  Rs=1e5  Cs=inf  Measurements=off
  Logical Operator : Logic  Inputs=1  AllPortsSameDT=off  OutDataTypeStr=boolean
  Logical Operator1 : Logic  Operator=NOT  Inputs=1  AllPortsSameDT=off  OutDataTypeStr=boolean
  Series RLC Branch : spsSeriesRLCBranchLib/Series RLC Branch  LConnTagsString=__new0  RConnTagsString=__new0  BranchType=C  Resistance=1  Inductance=1e-3  SetiL0=off  InitialCurrent=0  Capacitance=C0  Setx0=on  InitialVoltage=V0  Measurements=None
  Voltage Measurement : spsVoltageMeasurementLib/Voltage Measurement  PhasorSimulation=off  OutputType=Complex  PSBequivalent=0
  V+ : PMIOPort  Side=Left
  V- : PMIOPort  Port=2  Side=Left
  VC : Outport
  wires:
  Logical Operator1/1 -> IGBT/Diode1/1
  Voltage Measurement/1 -> VC/1
  Logical Operator/1 -> IGBT/Diode/1
  PWM/1 -> Logical Operator/1, Logical Operator1/1
  connections:
  Voltage Measurement/LConn1 -- Series RLC Branch/LConn1 -- IGBT/Diode/LConn1
  V+/RConn1 -- IGBT/Diode1/LConn1 -- IGBT/Diode/RConn1
  V-/RConn1 -- IGBT/Diode1/RConn1 -- Series RLC Branch/RConn1 -- Voltage Measurement/LConn2

== system MMC_Rectifier_NLM_2018/MMC  Rectifier/MMC3/MMC12 ==
  PWM : Inport
  IGBT/Diode : spsIGBTDiodeLib/IGBT//Diode  Ron=1e-3  Rs=1e5  Cs=inf  Measurements=off
  IGBT/Diode1 : spsIGBTDiodeLib/IGBT//Diode  Ron=1e-3  Rs=1e5  Cs=inf  Measurements=off
  Logical Operator : Logic  Inputs=1  AllPortsSameDT=off  OutDataTypeStr=boolean
  Logical Operator1 : Logic  Operator=NOT  Inputs=1  AllPortsSameDT=off  OutDataTypeStr=boolean
  Series RLC Branch : spsSeriesRLCBranchLib/Series RLC Branch  LConnTagsString=__new0  RConnTagsString=__new0  BranchType=C  Resistance=1  Inductance=1e-3  SetiL0=off  InitialCurrent=0  Capacitance=C0  Setx0=on  InitialVoltage=V0  Measurements=None
  Voltage Measurement : spsVoltageMeasurementLib/Voltage Measurement  PhasorSimulation=off  OutputType=Complex  PSBequivalent=0
  V+ : PMIOPort  Side=Left
  V- : PMIOPort  Port=2  Side=Left
  VC : Outport
  wires:
  Logical Operator1/1 -> IGBT/Diode1/1
  Voltage Measurement/1 -> VC/1
  Logical Operator/1 -> IGBT/Diode/1
  PWM/1 -> Logical Operator/1, Logical Operator1/1
  connections:
  Voltage Measurement/LConn1 -- Series RLC Branch/LConn1 -- IGBT/Diode/LConn1
  V+/RConn1 -- IGBT/Diode1/LConn1 -- IGBT/Diode/RConn1
  V-/RConn1 -- IGBT/Diode1/RConn1 -- Series RLC Branch/RConn1 -- Voltage Measurement/LConn2

== system MMC_Rectifier_NLM_2018/MMC  Rectifier/MMC3/MMC13 ==
  PWM : Inport
  IGBT/Diode : spsIGBTDiodeLib/IGBT//Diode  Ron=1e-3  Rs=1e5  Cs=inf  Measurements=off
  IGBT/Diode1 : spsIGBTDiodeLib/IGBT//Diode  Ron=1e-3  Rs=1e5  Cs=inf  Measurements=off
  Logical Operator : Logic  Inputs=1  AllPortsSameDT=off  OutDataTypeStr=boolean
  Logical Operator1 : Logic  Operator=NOT  Inputs=1  AllPortsSameDT=off  OutDataTypeStr=boolean
  Series RLC Branch : spsSeriesRLCBranchLib/Series RLC Branch  LConnTagsString=__new0  RConnTagsString=__new0  BranchType=C  Resistance=1  Inductance=1e-3  SetiL0=off  InitialCurrent=0  Capacitance=C0  Setx0=on  InitialVoltage=V0  Measurements=None
  Voltage Measurement : spsVoltageMeasurementLib/Voltage Measurement  PhasorSimulation=off  OutputType=Complex  PSBequivalent=0
  V+ : PMIOPort  Side=Left
  V- : PMIOPort  Port=2  Side=Left
  VC : Outport
  wires:
  PWM/1 -> Logical Operator1/1, Logical Operator/1
  Logical Operator/1 -> IGBT/Diode/1
  Voltage Measurement/1 -> VC/1
  Logical Operator1/1 -> IGBT/Diode1/1
  connections:
  Voltage Measurement/LConn2 -- Series RLC Branch/RConn1 -- IGBT/Diode1/RConn1 -- V-/RConn1
  IGBT/Diode/RConn1 -- IGBT/Diode1/LConn1 -- V+/RConn1
  IGBT/Diode/LConn1 -- Series RLC Branch/LConn1 -- Voltage Measurement/LConn1

== system MMC_Rectifier_NLM_2018/MMC  Rectifier/MMC3/MMC14 ==
  PWM : Inport
  IGBT/Diode : spsIGBTDiodeLib/IGBT//Diode  Ron=1e-3  Rs=1e5  Cs=inf  Measurements=off
  IGBT/Diode1 : spsIGBTDiodeLib/IGBT//Diode  Ron=1e-3  Rs=1e5  Cs=inf  Measurements=off
  Logical Operator : Logic  Inputs=1  AllPortsSameDT=off  OutDataTypeStr=boolean
  Logical Operator1 : Logic  Operator=NOT  Inputs=1  AllPortsSameDT=off  OutDataTypeStr=boolean
  Series RLC Branch : spsSeriesRLCBranchLib/Series RLC Branch  LConnTagsString=__new0  RConnTagsString=__new0  BranchType=C  Resistance=1  Inductance=1e-3  SetiL0=off  InitialCurrent=0  Capacitance=C0  Setx0=on  InitialVoltage=V0  Measurements=None
  Voltage Measurement : spsVoltageMeasurementLib/Voltage Measurement  PhasorSimulation=off  OutputType=Complex  PSBequivalent=0
  V+ : PMIOPort  Side=Left
  V- : PMIOPort  Port=2  Side=Left
  VC : Outport
  wires:
  Logical Operator1/1 -> IGBT/Diode1/1
  Voltage Measurement/1 -> VC/1
  Logical Operator/1 -> IGBT/Diode/1
  PWM/1 -> Logical Operator/1, Logical Operator1/1
  connections:
  IGBT/Diode/LConn1 -- Voltage Measurement/LConn1 -- Series RLC Branch/LConn1
  IGBT/Diode/RConn1 -- V+/RConn1 -- IGBT/Diode1/LConn1
  IGBT/Diode1/RConn1 -- V-/RConn1 -- Voltage Measurement/LConn2 -- Series RLC Branch/RConn1

== system MMC_Rectifier_NLM_2018/MMC  Rectifier/MMC3/MMC15 ==
  PWM : Inport
  IGBT/Diode : spsIGBTDiodeLib/IGBT//Diode  Ron=1e-3  Rs=1e5  Cs=inf  Measurements=off
  IGBT/Diode1 : spsIGBTDiodeLib/IGBT//Diode  Ron=1e-3  Rs=1e5  Cs=inf  Measurements=off
  Logical Operator : Logic  Inputs=1  AllPortsSameDT=off  OutDataTypeStr=boolean
  Logical Operator1 : Logic  Operator=NOT  Inputs=1  AllPortsSameDT=off  OutDataTypeStr=boolean
  Series RLC Branch : spsSeriesRLCBranchLib/Series RLC Branch  LConnTagsString=__new0  RConnTagsString=__new0  BranchType=C  Resistance=1  Inductance=1e-3  SetiL0=off  InitialCurrent=0  Capacitance=C0  Setx0=on  InitialVoltage=V0  Measurements=None
  Voltage Measurement : spsVoltageMeasurementLib/Voltage Measurement  PhasorSimulation=off  OutputType=Complex  PSBequivalent=0
  V+ : PMIOPort  Side=Left
  V- : PMIOPort  Port=2  Side=Left
  VC : Outport
  wires:
  PWM/1 -> Logical Operator1/1, Logical Operator/1
  Logical Operator/1 -> IGBT/Diode/1
  Voltage Measurement/1 -> VC/1
  Logical Operator1/1 -> IGBT/Diode1/1
  connections:
  Voltage Measurement/LConn2 -- Series RLC Branch/RConn1 -- IGBT/Diode1/RConn1 -- V-/RConn1
  IGBT/Diode/RConn1 -- IGBT/Diode1/LConn1 -- V+/RConn1
  IGBT/Diode/LConn1 -- Series RLC Branch/LConn1 -- Voltage Measurement/LConn1

== system MMC_Rectifier_NLM_2018/MMC  Rectifier/MMC3/MMC16 ==
  PWM : Inport
  IGBT/Diode : spsIGBTDiodeLib/IGBT//Diode  Ron=1e-3  Rs=1e5  Cs=inf  Measurements=off
  IGBT/Diode1 : spsIGBTDiodeLib/IGBT//Diode  Ron=1e-3  Rs=1e5  Cs=inf  Measurements=off
  Logical Operator : Logic  Inputs=1  AllPortsSameDT=off  OutDataTypeStr=boolean
  Logical Operator1 : Logic  Operator=NOT  Inputs=1  AllPortsSameDT=off  OutDataTypeStr=boolean
  Series RLC Branch : spsSeriesRLCBranchLib/Series RLC Branch  LConnTagsString=__new0  RConnTagsString=__new0  BranchType=C  Resistance=1  Inductance=1e-3  SetiL0=off  InitialCurrent=0  Capacitance=C0  Setx0=on  InitialVoltage=V0  Measurements=None
  Voltage Measurement : spsVoltageMeasurementLib/Voltage Measurement  PhasorSimulation=off  OutputType=Complex  PSBequivalent=0
  V+ : PMIOPort  Side=Left
  V- : PMIOPort  Port=2  Side=Left
  VC : Outport
  wires:
  PWM/1 -> Logical Operator1/1, Logical Operator/1
  Logical Operator/1 -> IGBT/Diode/1
  Voltage Measurement/1 -> VC/1
  Logical Operator1/1 -> IGBT/Diode1/1
  connections:
  Voltage Measurement/LConn2 -- Series RLC Branch/RConn1 -- IGBT/Diode1/RConn1 -- V-/RConn1
  IGBT/Diode/RConn1 -- IGBT/Diode1/LConn1 -- V+/RConn1
  IGBT/Diode/LConn1 -- Series RLC Branch/LConn1 -- Voltage Measurement/LConn1

== system MMC_Rectifier_NLM_2018/MMC  Rectifier/MMC3/MMC17 ==
  PWM : Inport
  IGBT/Diode : spsIGBTDiodeLib/IGBT//Diode  Ron=1e-3  Rs=1e5  Cs=inf  Measurements=off
  IGBT/Diode1 : spsIGBTDiodeLib/IGBT//Diode  Ron=1e-3  Rs=1e5  Cs=inf  Measurements=off
  Logical Operator : Logic  Inputs=1  AllPortsSameDT=off  OutDataTypeStr=boolean
  Logical Operator1 : Logic  Operator=NOT  Inputs=1  AllPortsSameDT=off  OutDataTypeStr=boolean
  Series RLC Branch : spsSeriesRLCBranchLib/Series RLC Branch  LConnTagsString=__new0  RConnTagsString=__new0  BranchType=C  Resistance=1  Inductance=1e-3  SetiL0=off  InitialCurrent=0  Capacitance=C0  Setx0=on  InitialVoltage=V0  Measurements=None
  Voltage Measurement : spsVoltageMeasurementLib/Voltage Measurement  PhasorSimulation=off  OutputType=Complex  PSBequivalent=0
  V+ : PMIOPort  Side=Left
  V- : PMIOPort  Port=2  Side=Left
  VC : Outport
  wires:
  Logical Operator1/1 -> IGBT/Diode1/1
  Voltage Measurement/1 -> VC/1
  Logical Operator/1 -> IGBT/Diode/1
  PWM/1 -> Logical Operator/1, Logical Operator1/1
  connections:
  Voltage Measurement/LConn1 -- Series RLC Branch/LConn1 -- IGBT/Diode/LConn1
  V+/RConn1 -- IGBT/Diode1/LConn1 -- IGBT/Diode/RConn1
  V-/RConn1 -- IGBT/Diode1/RConn1 -- Series RLC Branch/RConn1 -- Voltage Measurement/LConn2

== system MMC_Rectifier_NLM_2018/MMC  Rectifier/MMC3/MMC2 ==
  PWM : Inport
  IGBT/Diode : spsIGBTDiodeLib/IGBT//Diode  Ron=1e-3  Rs=1e5  Cs=inf  Measurements=off
  IGBT/Diode1 : spsIGBTDiodeLib/IGBT//Diode  Ron=1e-3  Rs=1e5  Cs=inf  Measurements=off
  Logical Operator : Logic  Inputs=1  AllPortsSameDT=off  OutDataTypeStr=boolean
  Logical Operator1 : Logic  Operator=NOT  Inputs=1  AllPortsSameDT=off  OutDataTypeStr=boolean
  Series RLC Branch : spsSeriesRLCBranchLib/Series RLC Branch  LConnTagsString=__new0  RConnTagsString=__new0  BranchType=C  Resistance=1  Inductance=1e-3  SetiL0=off  InitialCurrent=0  Capacitance=C0  Setx0=on  InitialVoltage=V0  Measurements=None
  Voltage Measurement : spsVoltageMeasurementLib/Voltage Measurement  PhasorSimulation=off  OutputType=Complex  PSBequivalent=0
  V+ : PMIOPort  Side=Left
  V- : PMIOPort  Port=2  Side=Left
  VC : Outport
  wires:
  PWM/1 -> Logical Operator1/1, Logical Operator/1
  Logical Operator/1 -> IGBT/Diode/1
  Voltage Measurement/1 -> VC/1
  Logical Operator1/1 -> IGBT/Diode1/1
  connections:
  Voltage Measurement/LConn2 -- Series RLC Branch/RConn1 -- IGBT/Diode1/RConn1 -- V-/RConn1
  IGBT/Diode/RConn1 -- IGBT/Diode1/LConn1 -- V+/RConn1
  IGBT/Diode/LConn1 -- Series RLC Branch/LConn1 -- Voltage Measurement/LConn1

== system MMC_Rectifier_NLM_2018/MMC  Rectifier/MMC3/MMC3 ==
  PWM : Inport
  IGBT/Diode : spsIGBTDiodeLib/IGBT//Diode  Ron=1e-3  Rs=1e5  Cs=inf  Measurements=off
  IGBT/Diode1 : spsIGBTDiodeLib/IGBT//Diode  Ron=1e-3  Rs=1e5  Cs=inf  Measurements=off
  Logical Operator : Logic  Inputs=1  AllPortsSameDT=off  OutDataTypeStr=boolean
  Logical Operator1 : Logic  Operator=NOT  Inputs=1  AllPortsSameDT=off  OutDataTypeStr=boolean
  Series RLC Branch : spsSeriesRLCBranchLib/Series RLC Branch  LConnTagsString=__new0  RConnTagsString=__new0  BranchType=C  Resistance=1  Inductance=1e-3  SetiL0=off  InitialCurrent=0  Capacitance=C0  Setx0=on  InitialVoltage=V0  Measurements=None
  Voltage Measurement : spsVoltageMeasurementLib/Voltage Measurement  PhasorSimulation=off  OutputType=Complex  PSBequivalent=0
  V+ : PMIOPort  Side=Left
  V- : PMIOPort  Port=2  Side=Left
  VC : Outport
  wires:
  Logical Operator1/1 -> IGBT/Diode1/1
  Voltage Measurement/1 -> VC/1
  Logical Operator/1 -> IGBT/Diode/1
  PWM/1 -> Logical Operator/1, Logical Operator1/1
  connections:
  Voltage Measurement/LConn1 -- Series RLC Branch/LConn1 -- IGBT/Diode/LConn1
  V+/RConn1 -- IGBT/Diode1/LConn1 -- IGBT/Diode/RConn1
  V-/RConn1 -- IGBT/Diode1/RConn1 -- Series RLC Branch/RConn1 -- Voltage Measurement/LConn2

== system MMC_Rectifier_NLM_2018/MMC  Rectifier/MMC3/MMC4 ==
  PWM : Inport
  IGBT/Diode : spsIGBTDiodeLib/IGBT//Diode  Ron=1e-3  Rs=1e5  Cs=inf  Measurements=off
  IGBT/Diode1 : spsIGBTDiodeLib/IGBT//Diode  Ron=1e-3  Rs=1e5  Cs=inf  Measurements=off
  Logical Operator : Logic  Inputs=1  AllPortsSameDT=off  OutDataTypeStr=boolean
  Logical Operator1 : Logic  Operator=NOT  Inputs=1  AllPortsSameDT=off  OutDataTypeStr=boolean
  Series RLC Branch : spsSeriesRLCBranchLib/Series RLC Branch  LConnTagsString=__new0  RConnTagsString=__new0  BranchType=C  Resistance=1  Inductance=1e-3  SetiL0=off  InitialCurrent=0  Capacitance=C0  Setx0=on  InitialVoltage=V0  Measurements=None
  Voltage Measurement : spsVoltageMeasurementLib/Voltage Measurement  PhasorSimulation=off  OutputType=Complex  PSBequivalent=0
  V+ : PMIOPort  Side=Left
  V- : PMIOPort  Port=2  Side=Left
  VC : Outport
  wires:
  Logical Operator1/1 -> IGBT/Diode1/1
  Voltage Measurement/1 -> VC/1
  Logical Operator/1 -> IGBT/Diode/1
  PWM/1 -> Logical Operator/1, Logical Operator1/1
  connections:
  Voltage Measurement/LConn1 -- Series RLC Branch/LConn1 -- IGBT/Diode/LConn1
  V+/RConn1 -- IGBT/Diode1/LConn1 -- IGBT/Diode/RConn1
  V-/RConn1 -- IGBT/Diode1/RConn1 -- Series RLC Branch/RConn1 -- Voltage Measurement/LConn2

== system MMC_Rectifier_NLM_2018/MMC  Rectifier/MMC3/MMC5 ==
  PWM : Inport
  IGBT/Diode : spsIGBTDiodeLib/IGBT//Diode  Ron=1e-3  Rs=1e5  Cs=inf  Measurements=off
  IGBT/Diode1 : spsIGBTDiodeLib/IGBT//Diode  Ron=1e-3  Rs=1e5  Cs=inf  Measurements=off
  Logical Operator : Logic  Inputs=1  AllPortsSameDT=off  OutDataTypeStr=boolean
  Logical Operator1 : Logic  Operator=NOT  Inputs=1  AllPortsSameDT=off  OutDataTypeStr=boolean
  Series RLC Branch : spsSeriesRLCBranchLib/Series RLC Branch  LConnTagsString=__new0  RConnTagsString=__new0  BranchType=C  Resistance=1  Inductance=1e-3  SetiL0=off  InitialCurrent=0  Capacitance=C0  Setx0=on  InitialVoltage=V0  Measurements=None
  Voltage Measurement : spsVoltageMeasurementLib/Voltage Measurement  PhasorSimulation=off  OutputType=Complex  PSBequivalent=0
  V+ : PMIOPort  Side=Left
  V- : PMIOPort  Port=2  Side=Left
  VC : Outport
  wires:
  PWM/1 -> Logical Operator1/1, Logical Operator/1
  Logical Operator/1 -> IGBT/Diode/1
  Voltage Measurement/1 -> VC/1
  Logical Operator1/1 -> IGBT/Diode1/1
  connections:
  Voltage Measurement/LConn2 -- Series RLC Branch/RConn1 -- IGBT/Diode1/RConn1 -- V-/RConn1
  IGBT/Diode/RConn1 -- IGBT/Diode1/LConn1 -- V+/RConn1
  IGBT/Diode/LConn1 -- Series RLC Branch/LConn1 -- Voltage Measurement/LConn1

== system MMC_Rectifier_NLM_2018/MMC  Rectifier/MMC3/MMC6 ==
  PWM : Inport
  IGBT/Diode : spsIGBTDiodeLib/IGBT//Diode  Ron=1e-3  Rs=1e5  Cs=inf  Measurements=off
  IGBT/Diode1 : spsIGBTDiodeLib/IGBT//Diode  Ron=1e-3  Rs=1e5  Cs=inf  Measurements=off
  Logical Operator : Logic  Inputs=1  AllPortsSameDT=off  OutDataTypeStr=boolean
  Logical Operator1 : Logic  Operator=NOT  Inputs=1  AllPortsSameDT=off  OutDataTypeStr=boolean
  Series RLC Branch : spsSeriesRLCBranchLib/Series RLC Branch  LConnTagsString=__new0  RConnTagsString=__new0  BranchType=C  Resistance=1  Inductance=1e-3  SetiL0=off  InitialCurrent=0  Capacitance=C0  Setx0=on  InitialVoltage=V0  Measurements=None
  Voltage Measurement : spsVoltageMeasurementLib/Voltage Measurement  PhasorSimulation=off  OutputType=Complex  PSBequivalent=0
  V+ : PMIOPort  Side=Left
  V- : PMIOPort  Port=2  Side=Left
  VC : Outport
  wires:
  PWM/1 -> Logical Operator1/1, Logical Operator/1
  Logical Operator/1 -> IGBT/Diode/1
  Voltage Measurement/1 -> VC/1
  Logical Operator1/1 -> IGBT/Diode1/1
  connections:
  Series RLC Branch/RConn1 -- Voltage Measurement/LConn2 -- V-/RConn1 -- IGBT/Diode1/RConn1
  IGBT/Diode1/LConn1 -- V+/RConn1 -- IGBT/Diode/RConn1
  Series RLC Branch/LConn1 -- Voltage Measurement/LConn1 -- IGBT/Diode/LConn1

== system MMC_Rectifier_NLM_2018/MMC  Rectifier/MMC3/MMC7 ==
  PWM : Inport
  IGBT/Diode : spsIGBTDiodeLib/IGBT//Diode  Ron=1e-3  Rs=1e5  Cs=inf  Measurements=off
  IGBT/Diode1 : spsIGBTDiodeLib/IGBT//Diode  Ron=1e-3  Rs=1e5  Cs=inf  Measurements=off
  Logical Operator : Logic  Inputs=1  AllPortsSameDT=off  OutDataTypeStr=boolean
  Logical Operator1 : Logic  Operator=NOT  Inputs=1  AllPortsSameDT=off  OutDataTypeStr=boolean
  Series RLC Branch : spsSeriesRLCBranchLib/Series RLC Branch  LConnTagsString=__new0  RConnTagsString=__new0  BranchType=C  Resistance=1  Inductance=1e-3  SetiL0=off  InitialCurrent=0  Capacitance=C0  Setx0=on  InitialVoltage=V0  Measurements=None
  Voltage Measurement : spsVoltageMeasurementLib/Voltage Measurement  PhasorSimulation=off  OutputType=Complex  PSBequivalent=0
  V+ : PMIOPort  Side=Left
  V- : PMIOPort  Port=2  Side=Left
  VC : Outport
  wires:
  Logical Operator1/1 -> IGBT/Diode1/1
  Voltage Measurement/1 -> VC/1
  Logical Operator/1 -> IGBT/Diode/1
  PWM/1 -> Logical Operator/1, Logical Operator1/1
  connections:
  Voltage Measurement/LConn1 -- Series RLC Branch/LConn1 -- IGBT/Diode/LConn1
  V+/RConn1 -- IGBT/Diode1/LConn1 -- IGBT/Diode/RConn1
  V-/RConn1 -- IGBT/Diode1/RConn1 -- Series RLC Branch/RConn1 -- Voltage Measurement/LConn2

== system MMC_Rectifier_NLM_2018/MMC  Rectifier/MMC3/MMC8 ==
  PWM : Inport
  IGBT/Diode : spsIGBTDiodeLib/IGBT//Diode  Ron=1e-3  Rs=1e5  Cs=inf  Measurements=off
  IGBT/Diode1 : spsIGBTDiodeLib/IGBT//Diode  Ron=1e-3  Rs=1e5  Cs=inf  Measurements=off
  Logical Operator : Logic  Inputs=1  AllPortsSameDT=off  OutDataTypeStr=boolean
  Logical Operator1 : Logic  Operator=NOT  Inputs=1  AllPortsSameDT=off  OutDataTypeStr=boolean
  Series RLC Branch : spsSeriesRLCBranchLib/Series RLC Branch  LConnTagsString=__new0  RConnTagsString=__new0  BranchType=C  Resistance=1  Inductance=1e-3  SetiL0=off  InitialCurrent=0  Capacitance=C0  Setx0=on  InitialVoltage=V0  Measurements=None
  Voltage Measurement : spsVoltageMeasurementLib/Voltage Measurement  PhasorSimulation=off  OutputType=Complex  PSBequivalent=0
  V+ : PMIOPort  Side=Left
  V- : PMIOPort  Port=2  Side=Left
  VC : Outport
  wires:
  Logical Operator1/1 -> IGBT/Diode1/1
  Voltage Measurement/1 -> VC/1
  Logical Operator/1 -> IGBT/Diode/1
  PWM/1 -> Logical Operator/1, Logical Operator1/1
  connections:
  Voltage Measurement/LConn1 -- Series RLC Branch/LConn1 -- IGBT/Diode/LConn1
  V+/RConn1 -- IGBT/Diode1/LConn1 -- IGBT/Diode/RConn1
  V-/RConn1 -- IGBT/Diode1/RConn1 -- Series RLC Branch/RConn1 -- Voltage Measurement/LConn2
